simulink model "ASM_Traffic_new"  (R2024a)
settings: Solver=ode1  StartTime=SIM.tstart.v  StopTime=SIM.tend.v  FixedStep=SIM.StepSize.v  RelTol=1e-3
PostLoadFcn:
  | if any(exist('dsrtsu_mdlpostloadfcn', 'file') ~= 0), dsrtsu_mdlpostloadfcn('Execute', bdroot); end
  | try, asm_mdl_postloadfcn(bdroot, 'UpdateModel', 3600); catch, disp(lasterr); end,
InitFcn:
  | , if any(exist('rtifpga_mdlclblib', 'file') ~= 0), rtifpga_mdlclblib('Init', bdroot); end,
  | , if any(exist('dsmpb_private', 'file') ~= 0), dsmpb_private('dsmpb_mdlclblib', 'Init', bdroot); end,
undefined symbols (not defined in the file): _to_, a0b2, ASM_BrakeHydraulics_DemoSystems, ASM_VehicleDynamics_DemoSystems, b98103fe8ad365046cd0, BrakeCircuit, CPT, Crankshaft, DiscIntNeverNeededParam, dsmsi, FinalDriveAssembly, MDL, ModeSignals, Pos_BrakePedal_Maneuver, rad, RefSignals, s_to_rpm, SIM, SoftECU, Suspension, Tire, Transmission
libraries: ASM_Traffic_lib x135, simulink x100, ASM_Utils_lib x77, ASM_VehicleDynamics_lib x70, ASM_Environment_lib x22, dsmpblib x20, dsmsilib x15, MDLD_Utils_lib x10, ASM_BrakeHydraulics_lib x3
(part 57 of 63)

== system ASM_Traffic_new/Environment/Sensors/PlantModel/Object_Sensor_3D/RadarEffects/Sensor2/RadarEffects ==
  Reset[] : Inport
  Sensor_Idx[] : Inport  Port=2
  Sensor_Data[] : Inport  Port=3
  Angle_Vehicle_CoorSys_E[x;y;z][deg] : Inport  Port=4
  Pos_Vehicle_CoorSys_E[x;y;z][m] : Inport  Port=5
  Angle_Sensor_CoorSys_V[x;y;z][deg] : Inport  Port=6
  Pos_Sensor_CoorSys_V[x;y;z][m] : Inport  Port=7
  Enable : EnablePort
  Bus Creator2 : BusCreator  Inputs=10
  Compare To Zero : simulink/Logic and Bit Operations/Compare To Zero  relop=>  OutDataTypeStr=boolean
  MODELDESK_GROUP : ASM_Utils_lib/ModelDeskInterface/MODELDESK_GROUP  MDLDGroup=Object Sensor 3D 2  ASMProperties=struct('Name','MODELDESK_GROUP','Version','1.0','Library','ASM_Utils_lib')
  RADAR_DETECTION_RANGE_2 : ASM_Traffic_lib/Sensors/RadarEffects/RADAR_DETECTION_RANGE  Tag=ASM_SUBCOMPONENT  Sw_Detection_Range_Enable=MDL.Traffic.Sensors.Radar_Detection_Range_2.Sw_Detection_Range_Enable  Const_Signal_Strength_Threshold=MDL.Traffic.Sensors.Radar_Detection_Range_2.Const_Signal_Strength_Threshold  Const_Attenuation=MDL.Traffic.Sensors.Radar_Detection_Range_2.Const_Attenuation  Map_Antenna_Gain=MDL.Traffic.Sensors.Radar_Detection_Range_2.Map_Antenna_Gain  ASMProperties=struct('Name','RADAR_DETECTION_RANGE','Version','1.0','Library','ASM_Traffic_lib')  ASMInstanceName=radar_detection_range  ASMInstanceID=2
      settings: AttributesFormatString=Instance Name: %<ASMInstanceName>\nInstance ID: %<ASMInstanceID>
  RADAR_MEASUREMENT_NOISE_2 : ASM_Traffic_lib/Sensors/RadarEffects/RADAR_MEASUREMENT_NOISE  Tag=ASM_SUBCOMPONENT  Sw_Measurement_Noise_Enable=MDL.Traffic.Sensors.Radar_Measurement_Noise_2.Sw_Measurement_Noise_Enable  Const_StdDev_Distance=MDL.Traffic.Sensors.Radar_Measurement_Noise_2.Const_StdDev_Distance  Const_StdDev_Angle_Hor=MDL.Traffic.Sensors.Radar_Measurement_Noise_2.Const_StdDev_Angle_Hor  Const_StdDev_Angle_Ver=MDL.Traffic.Sensors.Radar_Measurement_Noise_2.Const_StdDev_Angle_Ver  Const_StdDev_Velocity=MDL.Traffic.Sensors.Radar_Measurement_Noise_2.Const_StdDev_Velocity  Const_Seed_Distance=MDL.Traffic.Sensors.Radar_Measurement_Noise_2.Const_Seed_Distance  Const_Seed_Angle_Hor=MDL.Traffic.Sensors.Radar_Measurement_Noise_2.Const_Seed_Angle_Hor  Const_Seed_Angle_Ver=MDL.Traffic.Sensors.Radar_Measurement_Noise_2.Const_Seed_Angle_Ver  Const_Seed_Velocity=MDL.Traffic.Sensors.Radar_Measurement_Noise_2.Const_Seed_Velocity  Const_Output_Dimension_Objects=MDL.Traffic.Sensors.Radar_Measurement_Noise_2.Const_Output_Dimension_Objects  Const_Output_Dimension_Object_Points=MDL.Traffic.Sensors.Radar_Measurement_Noise_2.Const_Output_Dimension_Object_Points  SimStepSize=SIM.StepSize  ASMProperties=struct('Name','RADAR_MEASUREMENT_NOISE','Version','3.0','Library','ASM_Traffic_lib')  ASMInstanceName=radar_measurement_noise  ASMInstanceID=2
      settings: AttributesFormatString=Instance Name: %<ASMInstanceName>\nInstance ID: %<ASMInstanceID>
  RADAR_OUTPUT_SORT_2 : ASM_Traffic_lib/Sensors/RadarEffects/RADAR_OUTPUT_SORT  Tag=ASM_SUBCOMPONENT  Sw_Sort_Enable=MDL.Traffic.Sensors.Radar_Output_Sort_2.Sw_Sort_Enable  Sw_Sort_Attribute=MDL.Traffic.Sensors.Radar_Output_Sort_2.Sw_Sort_Attribute  Sw_Sort_Direction=MDL.Traffic.Sensors.Radar_Output_Sort_2.Sw_Sort_Direction  ASMProperties=struct('Name','RADAR_OUTPUT_SORT','Version','1.0','Library','ASM_Traffic_lib')  ASMInstanceName=radar_output_sort  ASMInstanceID=2
      settings: AttributesFormatString=Instance Name: %<ASMInstanceName>\nInstance ID: %<ASMInstanceID>
  RADAR_RCS_NOISE_2 : ASM_Traffic_lib/Sensors/RadarEffects/RADAR_RCS_NOISE  Tag=ASM_SUBCOMPONENT  Sw_RCS_Noise_Enable=MDL.Traffic.Sensors.Radar_RCS_Noise_2.Sw_RCS_Noise_Enable  Const_StdDev_RCS_Noise=MDL.Traffic.Sensors.Radar_RCS_Noise_2.Const_StdDev_RCS_Noise  Const_Seed_RCS_Noise=MDL.Traffic.Sensors.Radar_RCS_Noise_2.Const_Seed_RCS_Noise  Const_Output_Dimension_Objects=MDL.Traffic.Sensors.Radar_RCS_Noise_2.Const_Output_Dimension_Objects  Const_Output_Dimension_Object_Points=MDL.Traffic.Sensors.Radar_RCS_Noise_2.Const_Output_Dimension_Object_Points  SimStepSize=SIM.StepSize  ASMProperties=struct('Name','RADAR_RCS_NOISE','Version','3.0','Library','ASM_Traffic_lib')  ASMInstanceName=radar_rcs_noise  ASMInstanceID=2
      settings: AttributesFormatString=Instance Name: %<ASMInstanceName>\nInstance ID: %<ASMInstanceID>
  RADAR_REFLECTION_POINTS_2 : ASM_Traffic_lib/Sensors/RadarEffects/RADAR_REFLECTION_POINTS  Const_Output_Dimension_Objects=MDL.Traffic.Sensors.RadarReflectionPoints_2.Const_Output_Dimension_Objects  Const_Output_Dimension_Object_Points=MDL.Traffic.Sensors.RadarReflectionPoints_2.Const_Output_Dimension_Object_Points  ASMProperties=struct('Name','RADAR_REFLECTION_POINTS','Version','1.0','Library','ASM_Traffic_lib')  ASMInstanceName=radar_reflection_points  ASMInstanceID=2
  RADAR_REFLECTION_POINTS_COORDINATES_2 : ASM_Traffic_lib/Sensors/RadarEffects/RADAR_REFLECTION_POINTS_COORDINATES  ASMProperties=struct('Name','RADAR_REFLECTION_POINTS_COORDINATES','Version','1.0','Library','ASM_Traffic_lib')  ASMInstanceName=radar_reflection_points_coordinates  ASMInstanceID=1
  RADAR_RESOLUTION_CELLS_2 : ASM_Traffic_lib/Sensors/RadarEffects/RADAR_RESOLUTION_CELLS  Tag=ASM_SUBCOMPONENT  Sw_Resolution_Cells_Enable=MDL.Traffic.Sensors.Radar_Resolution_Cells_2.Sw_Resolution_Cells_Enable  Sw_Distance_Resolution_Enable=MDL.Traffic.Sensors.Radar_Resolution_Cells_2.Sw_Distance_Resolution_Enable  Sw_Angle_Hor_Resolution_Enable=MDL.Traffic.Sensors.Radar_Resolution_Cells_2.Sw_Angle_Hor_Resolution_Enable  Sw_Angle_Ver_Resolution_Enable=MDL.Traffic.Sensors.Radar_Resolution_Cells_2.Sw_Angle_Ver_Resolution_Enable  Sw_Velocity_Resolution_Enable=MDL.Traffic.Sensors.Radar_Resolution_Cells_2.Sw_Velocity_Resolution_Enable  Const_Distance_Resolution=MDL.Traffic.Sensors.Radar_Resolution_Cells_2.Const_Distance_Resolution  Const_Angle_Hor_Resolution=MDL.Traffic.Sensors.Radar_Resolution_Cells_2.Const_Angle_Hor_Resolution  Const_Angle_Ver_Resolution=MDL.Traffic.Sensors.Radar_Resolution_Cells_2.Const_Angle_Ver_Resolution  Const_Velocity_Resolution=MDL.Traffic.Sensors.Radar_Resolution_Cells_2.Const_Velocity_Resolution  ASMProperties=struct('Name','RADAR_RESOLUTION_CELLS','Version','1.0','Library','ASM_Traffic_lib')  ASMInstanceName=radar_resolution_cells  ASMInstanceID=2
      settings: AttributesFormatString=Instance Name: %<ASMInstanceName>\nInstance ID: %<ASMInstanceID>
  Terminator{1..6,18} (7 alike) : Terminator
  RadarEffect_Signals[] : Outport  OutputWhenDisabled=reset  InitialOutput=[0]  VectorParamsAs1DForOutWhenUnconnected=off
  wires:
  RADAR_DETECTION_RANGE_2/6 -> RADAR_MEASUREMENT_NOISE_2/6
  RADAR_DETECTION_RANGE_2/5 -> RADAR_MEASUREMENT_NOISE_2/5
  RADAR_DETECTION_RANGE_2/4 -> RADAR_MEASUREMENT_NOISE_2/4
  RADAR_DETECTION_RANGE_2/3 -> RADAR_MEASUREMENT_NOISE_2/3
  RADAR_DETECTION_RANGE_2/2 -> RADAR_OUTPUT_SORT_2/1, RADAR_MEASUREMENT_NOISE_2/2
  Reset[]/1 -> RADAR_RCS_NOISE_2/1, RADAR_MEASUREMENT_NOISE_2/1
  RADAR_REFLECTION_POINTS_2/7 -> RADAR_RCS_NOISE_2/3
  RADAR_OUTPUT_SORT_2/6 -> RADAR_REFLECTION_POINTS_COORDINATES_2/8, Bus Creator2/5  "Angle_Ver_CoorSys_S[deg]"
  RADAR_OUTPUT_SORT_2/9 -> Bus Creator2/8  "Object_Type[]"
  RADAR_OUTPUT_SORT_2/5 -> RADAR_REFLECTION_POINTS_COORDINATES_2/7, Bus Creator2/4  "Angle_Hor_CoorSys_S[deg]"
  RADAR_REFLECTION_POINTS_COORDINATES_2/3 -> Bus Creator2/10  "Pos_ObjectPoint_CoorSys_S[x;y;z][m]"
  RADAR_OUTPUT_SORT_2/2 -> Compare To Zero/1, Bus Creator2/1  "ID[]"
  RADAR_OUTPUT_SORT_2/4 -> Bus Creator2/3  "v_CoorSys_S[m|s]"
  RADAR_OUTPUT_SORT_2/7 -> Bus Creator2/6  "RCS[dBm2]"
  RADAR_REFLECTION_POINTS_COORDINATES_2/2 -> Bus Creator2/9  "Pos_ObjectPoint_CoorSys_E[x;y;z][m]"
  RADAR_OUTPUT_SORT_2/8 -> Bus Creator2/7  "Object_ID[]"
  RADAR_OUTPUT_SORT_2/3 -> RADAR_REFLECTION_POINTS_COORDINATES_2/6, Bus Creator2/2  "Dist_CoorSys_S[m]"
  Compare To Zero/1 -> RADAR_REFLECTION_POINTS_COORDINATES_2/5
  RADAR_REFLECTION_POINTS_COORDINATES_2/1 -> Terminator6/1
  Pos_Sensor_CoorSys_V[x;y;z][m]/1 -> RADAR_REFLECTION_POINTS_COORDINATES_2/4
  Angle_Sensor_CoorSys_V[x;y;z][deg]/1 -> RADAR_REFLECTION_POINTS_COORDINATES_2/3
  Pos_Vehicle_CoorSys_E[x;y;z][m]/1 -> RADAR_REFLECTION_POINTS_COORDINATES_2/2
  Angle_Vehicle_CoorSys_E[x;y;z][deg]/1 -> RADAR_REFLECTION_POINTS_COORDINATES_2/1
  Bus Creator2/1 -> RadarEffect_Signals[]/1
  Sensor_Data[]/1 -> RADAR_REFLECTION_POINTS_2/2
  RADAR_RESOLUTION_CELLS_2/5 -> RADAR_DETECTION_RANGE_2/4
  RADAR_RESOLUTION_CELLS_2/8 -> RADAR_DETECTION_RANGE_2/7
  RADAR_MEASUREMENT_NOISE_2/5 -> RADAR_OUTPUT_SORT_2/5
  RADAR_MEASUREMENT_NOISE_2/1 -> Terminator4/1
  RADAR_OUTPUT_SORT_2/1 -> Terminator5/1
  RADAR_REFLECTION_POINTS_2/3 -> RADAR_RESOLUTION_CELLS_2/2
  RADAR_DETECTION_RANGE_2/9 -> RADAR_OUTPUT_SORT_2/8
  RADAR_RESOLUTION_CELLS_2/3 -> RADAR_DETECTION_RANGE_2/2
  RADAR_REFLECTION_POINTS_2/4 -> RADAR_RESOLUTION_CELLS_2/3
  Sensor_Idx[]/1 -> RADAR_REFLECTION_POINTS_2/1
  RADAR_DETECTION_RANGE_2/1 -> Terminator2/1
  RADAR_REFLECTION_POINTS_2/2 -> RADAR_RCS_NOISE_2/2, RADAR_RESOLUTION_CELLS_2/1
  RADAR_DETECTION_RANGE_2/7 -> RADAR_OUTPUT_SORT_2/6
  RADAR_REFLECTION_POINTS_2/9 -> RADAR_RESOLUTION_CELLS_2/8
  RADAR_DETECTION_RANGE_2/8 -> RADAR_OUTPUT_SORT_2/7
  RADAR_RESOLUTION_CELLS_2/1 -> Terminator18/1
  RADAR_REFLECTION_POINTS_2/6 -> RADAR_RESOLUTION_CELLS_2/5
  RADAR_MEASUREMENT_NOISE_2/3 -> RADAR_OUTPUT_SORT_2/3
  RADAR_MEASUREMENT_NOISE_2/4 -> RADAR_OUTPUT_SORT_2/4
  RADAR_RESOLUTION_CELLS_2/9 -> RADAR_DETECTION_RANGE_2/8
  RADAR_REFLECTION_POINTS_2/8 -> RADAR_RESOLUTION_CELLS_2/7
  RADAR_MEASUREMENT_NOISE_2/2 -> RADAR_OUTPUT_SORT_2/2
  RADAR_RESOLUTION_CELLS_2/2 -> RADAR_DETECTION_RANGE_2/1
  RADAR_RESOLUTION_CELLS_2/7 -> RADAR_DETECTION_RANGE_2/6
  RADAR_RESOLUTION_CELLS_2/6 -> RADAR_DETECTION_RANGE_2/5
  RADAR_RCS_NOISE_2/1 -> Terminator1/1
  RADAR_REFLECTION_POINTS_2/5 -> RADAR_RESOLUTION_CELLS_2/4
  RADAR_REFLECTION_POINTS_2/1 -> Terminator3/1
  RADAR_RESOLUTION_CELLS_2/4 -> RADAR_DETECTION_RANGE_2/3
  RADAR_RCS_NOISE_2/2 -> RADAR_RESOLUTION_CELLS_2/6

== system ASM_Traffic_new/Environment/Sensors/PlantModel/Object_Sensor_3D/RadarEffects/Sensor2/RadarEffectsOutput ==
  SensorScheudlingEnable[0|1] : Inport
  SensorActive : Inport  Port=2
  SensorEnable[0|1] : Inport  Port=3
  DelayPulse[0|1] : Inport  Port=4
  RadarEffect_Signals_In[] : Inport  Port=5
  HoldSignals : Subsystem
  Logical Operator2 : Logic  Operator=OR  AllPortsSameDT=off  OutDataTypeStr=boolean
  RADAR_SIGNALS_DELAY_2 : ASM_Traffic_lib/Sensors/RadarEffects/RADAR_SIGNALS_DELAY  ASMProperties=struct('Name','RADAR_SIGNALS_DELAY','Version','1.0','Library','ASM_Traffic_lib')  ASMInstanceName=radar_signals_delay  ASMInstanceID=1
  ResetPulse : Subsystem
  SignalBus : Subsystem
  RadarEffect_Signals_Out[] : Outport  VectorParamsAs1DForOutWhenUnconnected=off
  wires:
  Logical Operator2/1 -> HoldSignals/Enable
  SensorEnable[0|1]/1 -> Logical Operator2/2
  SensorScheudlingEnable[0|1]/1 -> ResetPulse/1(Enable[0|1])
  HoldSignals/1(RadarEffect_Signals_Out[]) -> RADAR_SIGNALS_DELAY_2/3
  RadarEffect_Signals_In[]/1 -> HoldSignals/2(RadarEffect_Signals_In[])
  SensorActive/1 -> ResetPulse/2(SensorActive[0|1])
  DelayPulse[0|1]/1 -> RADAR_SIGNALS_DELAY_2/2
  ResetPulse/1(ResetPulse[0|1]) -> HoldSignals/1(ResetPulse[0|1]), Logical Operator2/1, RADAR_SIGNALS_DELAY_2/1
  SignalBus/1(RadarEffect_Signals_Out[]) -> RadarEffect_Signals_Out[]/1
  RADAR_SIGNALS_DELAY_2/1 -> SignalBus/1(RadarEffect_Signals_In[])

== system ASM_Traffic_new/Environment/Sensors/PlantModel/Object_Sensor_3D/RadarEffects/Sensor3/RadarEffects ==
  Reset[] : Inport
  Sensor_Idx[] : Inport  Port=2
  Sensor_Data[] : Inport  Port=3
  Angle_Vehicle_CoorSys_E[x;y;z][deg] : Inport  Port=4
  Pos_Vehicle_CoorSys_E[x;y;z][m] : Inport  Port=5
  Angle_Sensor_CoorSys_V[x;y;z][deg] : Inport  Port=6
  Pos_Sensor_CoorSys_V[x;y;z][m] : Inport  Port=7
  Enable : EnablePort
  Bus Creator2 : BusCreator  Inputs=10
  Compare To Zero : simulink/Logic and Bit Operations/Compare To Zero  relop=>  OutDataTypeStr=boolean
  MODELDESK_GROUP : ASM_Utils_lib/ModelDeskInterface/MODELDESK_GROUP  MDLDGroup=Object Sensor 3D 3  ASMProperties=struct('Name','MODELDESK_GROUP','Version','1.0','Library','ASM_Utils_lib')
  RADAR_DETECTION_RANGE_3 : ASM_Traffic_lib/Sensors/RadarEffects/RADAR_DETECTION_RANGE  Tag=ASM_SUBCOMPONENT  Sw_Detection_Range_Enable=MDL.Traffic.Sensors.Radar_Detection_Range_3.Sw_Detection_Range_Enable  Const_Signal_Strength_Threshold=MDL.Traffic.Sensors.Radar_Detection_Range_3.Const_Signal_Strength_Threshold  Const_Attenuation=MDL.Traffic.Sensors.Radar_Detection_Range_3.Const_Attenuation  Map_Antenna_Gain=MDL.Traffic.Sensors.Radar_Detection_Range_3.Map_Antenna_Gain  ASMProperties=struct('Name','RADAR_DETECTION_RANGE','Version','1.0','Library','ASM_Traffic_lib')  ASMInstanceName=radar_detection_range  ASMInstanceID=3
      settings: AttributesFormatString=Instance Name: %<ASMInstanceName>\nInstance ID: %<ASMInstanceID>
  RADAR_MEASUREMENT_NOISE_3 : ASM_Traffic_lib/Sensors/RadarEffects/RADAR_MEASUREMENT_NOISE  Tag=ASM_SUBCOMPONENT  Sw_Measurement_Noise_Enable=MDL.Traffic.Sensors.Radar_Measurement_Noise_3.Sw_Measurement_Noise_Enable  Const_StdDev_Distance=MDL.Traffic.Sensors.Radar_Measurement_Noise_3.Const_StdDev_Distance  Const_StdDev_Angle_Hor=MDL.Traffic.Sensors.Radar_Measurement_Noise_3.Const_StdDev_Angle_Hor  Const_StdDev_Angle_Ver=MDL.Traffic.Sensors.Radar_Measurement_Noise_3.Const_StdDev_Angle_Ver  Const_StdDev_Velocity=MDL.Traffic.Sensors.Radar_Measurement_Noise_3.Const_StdDev_Velocity  Const_Seed_Distance=MDL.Traffic.Sensors.Radar_Measurement_Noise_3.Const_Seed_Distance  Const_Seed_Angle_Hor=MDL.Traffic.Sensors.Radar_Measurement_Noise_3.Const_Seed_Angle_Hor  Const_Seed_Angle_Ver=MDL.Traffic.Sensors.Radar_Measurement_Noise_3.Const_Seed_Angle_Ver  Const_Seed_Velocity=MDL.Traffic.Sensors.Radar_Measurement_Noise_3.Const_Seed_Velocity  Const_Output_Dimension_Objects=MDL.Traffic.Sensors.Radar_Measurement_Noise_3.Const_Output_Dimension_Objects  Const_Output_Dimension_Object_Points=MDL.Traffic.Sensors.Radar_Measurement_Noise_3.Const_Output_Dimension_Object_Points  SimStepSize=SIM.StepSize  ASMProperties=struct('Name','RADAR_MEASUREMENT_NOISE','Version','3.0','Library','ASM_Traffic_lib')  ASMInstanceName=radar_measurement_noise  ASMInstanceID=3
      settings: AttributesFormatString=Instance Name: %<ASMInstanceName>\nInstance ID: %<ASMInstanceID>
  RADAR_OUTPUT_SORT_3 : ASM_Traffic_lib/Sensors/RadarEffects/RADAR_OUTPUT_SORT  Tag=ASM_SUBCOMPONENT  Sw_Sort_Enable=MDL.Traffic.Sensors.Radar_Output_Sort_3.Sw_Sort_Enable  Sw_Sort_Attribute=MDL.Traffic.Sensors.Radar_Output_Sort_3.Sw_Sort_Attribute  Sw_Sort_Direction=MDL.Traffic.Sensors.Radar_Output_Sort_3.Sw_Sort_Direction  ASMProperties=struct('Name','RADAR_OUTPUT_SORT','Version','1.0','Library','ASM_Traffic_lib')  ASMInstanceName=radar_output_sort  ASMInstanceID=3
      settings: AttributesFormatString=Instance Name: %<ASMInstanceName>\nInstance ID: %<ASMInstanceID>
  RADAR_RCS_NOISE_3 : ASM_Traffic_lib/Sensors/RadarEffects/RADAR_RCS_NOISE  Tag=ASM_SUBCOMPONENT  Sw_RCS_Noise_Enable=MDL.Traffic.Sensors.Radar_RCS_Noise_3.Sw_RCS_Noise_Enable  Const_StdDev_RCS_Noise=MDL.Traffic.Sensors.Radar_RCS_Noise_3.Const_StdDev_RCS_Noise  Const_Seed_RCS_Noise=MDL.Traffic.Sensors.Radar_RCS_Noise_3.Const_Seed_RCS_Noise  Const_Output_Dimension_Objects=MDL.Traffic.Sensors.Radar_RCS_Noise_3.Const_Output_Dimension_Objects  Const_Output_Dimension_Object_Points=MDL.Traffic.Sensors.Radar_RCS_Noise_3.Const_Output_Dimension_Object_Points  SimStepSize=SIM.StepSize  ASMProperties=struct('Name','RADAR_RCS_NOISE','Version','3.0','Library','ASM_Traffic_lib')  ASMInstanceName=radar_rcs_noise  ASMInstanceID=3
      settings: AttributesFormatString=Instance Name: %<ASMInstanceName>\nInstance ID: %<ASMInstanceID>
  RADAR_REFLECTION_POINTS_3 : ASM_Traffic_lib/Sensors/RadarEffects/RADAR_REFLECTION_POINTS  Const_Output_Dimension_Objects=MDL.Traffic.Sensors.RadarReflectionPoints_3.Const_Output_Dimension_Objects  Const_Output_Dimension_Object_Points=MDL.Traffic.Sensors.RadarReflectionPoints_3.Const_Output_Dimension_Object_Points  ASMProperties=struct('Name','RADAR_REFLECTION_POINTS','Version','1.0','Library','ASM_Traffic_lib')  ASMInstanceName=radar_reflection_points  ASMInstanceID=3
  RADAR_REFLECTION_POINTS_COORDINATES_3 : ASM_Traffic_lib/Sensors/RadarEffects/RADAR_REFLECTION_POINTS_COORDINATES  ASMProperties=struct('Name','RADAR_REFLECTION_POINTS_COORDINATES','Version','1.0','Library','ASM_Traffic_lib')  ASMInstanceName=radar_reflection_points_coordinates  ASMInstanceID=1
  RADAR_RESOLUTION_CELLS_3 : ASM_Traffic_lib/Sensors/RadarEffects/RADAR_RESOLUTION_CELLS  Tag=ASM_SUBCOMPONENT  Sw_Resolution_Cells_Enable=MDL.Traffic.Sensors.Radar_Resolution_Cells_3.Sw_Resolution_Cells_Enable  Sw_Distance_Resolution_Enable=MDL.Traffic.Sensors.Radar_Resolution_Cells_3.Sw_Distance_Resolution_Enable  Sw_Angle_Hor_Resolution_Enable=MDL.Traffic.Sensors.Radar_Resolution_Cells_3.Sw_Angle_Hor_Resolution_Enable  Sw_Angle_Ver_Resolution_Enable=MDL.Traffic.Sensors.Radar_Resolution_Cells_3.Sw_Angle_Ver_Resolution_Enable  Sw_Velocity_Resolution_Enable=MDL.Traffic.Sensors.Radar_Resolution_Cells_3.Sw_Velocity_Resolution_Enable  Const_Distance_Resolution=MDL.Traffic.Sensors.Radar_Resolution_Cells_3.Const_Distance_Resolution  Const_Angle_Hor_Resolution=MDL.Traffic.Sensors.Radar_Resolution_Cells_3.Const_Angle_Hor_Resolution  Const_Angle_Ver_Resolution=MDL.Traffic.Sensors.Radar_Resolution_Cells_3.Const_Angle_Ver_Resolution  Const_Velocity_Resolution=MDL.Traffic.Sensors.Radar_Resolution_Cells_3.Const_Velocity_Resolution  ASMProperties=struct('Name','RADAR_RESOLUTION_CELLS','Version','1.0','Library','ASM_Traffic_lib')  ASMInstanceName=radar_resolution_cells  ASMInstanceID=3
      settings: AttributesFormatString=Instance Name: %<ASMInstanceName>\nInstance ID: %<ASMInstanceID>
  Terminator{1..6,18} (7 alike) : Terminator
  RadarEffect_Signals[] : Outport  OutputWhenDisabled=reset  InitialOutput=[0]  VectorParamsAs1DForOutWhenUnconnected=off
  wires:
  RADAR_DETECTION_RANGE_3/6 -> RADAR_MEASUREMENT_NOISE_3/6
  RADAR_DETECTION_RANGE_3/5 -> RADAR_MEASUREMENT_NOISE_3/5
  RADAR_DETECTION_RANGE_3/4 -> RADAR_MEASUREMENT_NOISE_3/4
  RADAR_DETECTION_RANGE_3/3 -> RADAR_MEASUREMENT_NOISE_3/3
  RADAR_DETECTION_RANGE_3/2 -> RADAR_MEASUREMENT_NOISE_3/2, RADAR_OUTPUT_SORT_3/1
  Reset[]/1 -> RADAR_RCS_NOISE_3/1, RADAR_MEASUREMENT_NOISE_3/1
  RADAR_REFLECTION_POINTS_3/7 -> RADAR_RCS_NOISE_3/3
  RADAR_REFLECTION_POINTS_COORDINATES_3/2 -> Bus Creator2/9  "Pos_ObjectPoint_CoorSys_E[x;y;z][m]"
  RADAR_OUTPUT_SORT_3/7 -> Bus Creator2/6  "RCS[dBm2]"
  RADAR_OUTPUT_SORT_3/9 -> Bus Creator2/8  "Object_Type[]"
  RADAR_OUTPUT_SORT_3/8 -> Bus Creator2/7  "Object_ID[]"
  RADAR_OUTPUT_SORT_3/3 -> RADAR_REFLECTION_POINTS_COORDINATES_3/6, Bus Creator2/2  "Dist_CoorSys_S[m]"
  RADAR_OUTPUT_SORT_3/4 -> Bus Creator2/3  "v_CoorSys_S[m|s]"
  RADAR_OUTPUT_SORT_3/6 -> RADAR_REFLECTION_POINTS_COORDINATES_3/8, Bus Creator2/5  "Angle_Ver_CoorSys_S[deg]"
  RADAR_OUTPUT_SORT_3/5 -> RADAR_REFLECTION_POINTS_COORDINATES_3/7, Bus Creator2/4  "Angle_Hor_CoorSys_S[deg]"
  RADAR_REFLECTION_POINTS_COORDINATES_3/3 -> Bus Creator2/10  "Pos_ObjectPoint_CoorSys_S[x;y;z][m]"
  RADAR_OUTPUT_SORT_3/2 -> Compare To Zero/1, Bus Creator2/1  "ID[]"
  Compare To Zero/1 -> RADAR_REFLECTION_POINTS_COORDINATES_3/5
  Pos_Sensor_CoorSys_V[x;y;z][m]/1 -> RADAR_REFLECTION_POINTS_COORDINATES_3/4
  Angle_Sensor_CoorSys_V[x;y;z][deg]/1 -> RADAR_REFLECTION_POINTS_COORDINATES_3/3
  Pos_Vehicle_CoorSys_E[x;y;z][m]/1 -> RADAR_REFLECTION_POINTS_COORDINATES_3/2
  Angle_Vehicle_CoorSys_E[x;y;z][deg]/1 -> RADAR_REFLECTION_POINTS_COORDINATES_3/1
  RADAR_REFLECTION_POINTS_COORDINATES_3/1 -> Terminator6/1
  Bus Creator2/1 -> RadarEffect_Signals[]/1
  RADAR_MEASUREMENT_NOISE_3/5 -> RADAR_OUTPUT_SORT_3/5
  Sensor_Data[]/1 -> RADAR_REFLECTION_POINTS_3/2
  RADAR_RESOLUTION_CELLS_3/7 -> RADAR_DETECTION_RANGE_3/6
  RADAR_REFLECTION_POINTS_3/9 -> RADAR_RESOLUTION_CELLS_3/8
  RADAR_RESOLUTION_CELLS_3/1 -> Terminator18/1
  RADAR_DETECTION_RANGE_3/8 -> RADAR_OUTPUT_SORT_3/7
  RADAR_RESOLUTION_CELLS_3/6 -> RADAR_DETECTION_RANGE_3/5
  RADAR_OUTPUT_SORT_3/1 -> Terminator5/1
  RADAR_MEASUREMENT_NOISE_3/3 -> RADAR_OUTPUT_SORT_3/3
  RADAR_RCS_NOISE_3/2 -> RADAR_RESOLUTION_CELLS_3/6
  RADAR_MEASUREMENT_NOISE_3/1 -> Terminator4/1
  RADAR_DETECTION_RANGE_3/7 -> RADAR_OUTPUT_SORT_3/6
  RADAR_DETECTION_RANGE_3/9 -> RADAR_OUTPUT_SORT_3/8
  RADAR_REFLECTION_POINTS_3/3 -> RADAR_RESOLUTION_CELLS_3/2
  RADAR_RESOLUTION_CELLS_3/9 -> RADAR_DETECTION_RANGE_3/8
  RADAR_REFLECTION_POINTS_3/5 -> RADAR_RESOLUTION_CELLS_3/4
  RADAR_RESOLUTION_CELLS_3/5 -> RADAR_DETECTION_RANGE_3/4
  RADAR_RESOLUTION_CELLS_3/4 -> RADAR_DETECTION_RANGE_3/3
  RADAR_MEASUREMENT_NOISE_3/2 -> RADAR_OUTPUT_SORT_3/2
  RADAR_REFLECTION_POINTS_3/4 -> RADAR_RESOLUTION_CELLS_3/3
  RADAR_REFLECTION_POINTS_3/8 -> RADAR_RESOLUTION_CELLS_3/7
  RADAR_RESOLUTION_CELLS_3/8 -> RADAR_DETECTION_RANGE_3/7
  RADAR_MEASUREMENT_NOISE_3/4 -> RADAR_OUTPUT_SORT_3/4
  RADAR_DETECTION_RANGE_3/1 -> Terminator2/1
  Sensor_Idx[]/1 -> RADAR_REFLECTION_POINTS_3/1
  RADAR_REFLECTION_POINTS_3/2 -> RADAR_RCS_NOISE_3/2, RADAR_RESOLUTION_CELLS_3/1
  RADAR_RESOLUTION_CELLS_3/2 -> RADAR_DETECTION_RANGE_3/1
  RADAR_REFLECTION_POINTS_3/1 -> Terminator3/1
  RADAR_RCS_NOISE_3/1 -> Terminator1/1
  RADAR_RESOLUTION_CELLS_3/3 -> RADAR_DETECTION_RANGE_3/2
  RADAR_REFLECTION_POINTS_3/6 -> RADAR_RESOLUTION_CELLS_3/5

== system ASM_Traffic_new/Environment/Sensors/PlantModel/Object_Sensor_3D/RadarEffects/Sensor3/RadarEffectsOutput ==
  SensorSchedulingEnable[0|1] : Inport
  SensorActive[0|1] : Inport  Port=2
  SensorEnable[0|1] : Inport  Port=3
  DelayPulse[0|1] : Inport  Port=4
  RadarEffect_Signals_In[] : Inport  Port=5
  HoldSignals : Subsystem
  Logical Operator1 : Logic  Operator=OR  AllPortsSameDT=off  OutDataTypeStr=boolean
  RADAR_SIGNALS_DELAY_3 : ASM_Traffic_lib/Sensors/RadarEffects/RADAR_SIGNALS_DELAY  ASMProperties=struct('Name','RADAR_SIGNALS_DELAY','Version','1.0','Library','ASM_Traffic_lib')  ASMInstanceName=radar_signals_delay  ASMInstanceID=1
  ResetPulse : Subsystem
  SignalBus : Subsystem
  RadarEffect_Signals_Out[] : Outport  VectorParamsAs1DForOutWhenUnconnected=off
  wires:
  SensorEnable[0|1]/1 -> Logical Operator1/2
  SensorActive[0|1]/1 -> ResetPulse/2(SensorActive[0|1])
  HoldSignals/1(RadarEffect_Signals_Out[]) -> RADAR_SIGNALS_DELAY_3/3
  ResetPulse/1(ResetPulse[0|1]) -> HoldSignals/1(ResetPulse[0|1]), Logical Operator1/1, RADAR_SIGNALS_DELAY_3/1
  SensorSchedulingEnable[0|1]/1 -> ResetPulse/1(Enable[0|1])
  Logical Operator1/1 -> HoldSignals/Enable
  SignalBus/1(RadarEffect_Signals_Out[]) -> RadarEffect_Signals_Out[]/1
  RadarEffect_Signals_In[]/1 -> HoldSignals/2(RadarEffect_Signals_In[])
  DelayPulse[0|1]/1 -> RADAR_SIGNALS_DELAY_3/2
  RADAR_SIGNALS_DELAY_3/1 -> SignalBus/1(RadarEffect_Signals_In[])

== system ASM_Traffic_new/Environment/Sensors/UserInterface/DISP_Plant/Object_Sensor_2D/IdxSelect_2DSensor/Scopezone_Element_Data_Selection1 ==
  Scopezone_El_Idx[1_60] : Inport
  Flag_Object_In_Scope[0Out|1In] : Inport  Port=2
  Flag_Sensor_Apex_In_Object[0Out|1In] : Inport  Port=3
  Angle_Hor_Rel[deg] : Inport  Port=4
  Object_ID[] : Inport  Port=5
  Object_Type[] : Inport  Port=6
  Distance[m] : Inport  Port=7
  v_Rel[m|s] : Inport  Port=8
  a_Rel[m|s2] : Inport  Port=9
  Height_Min[m] : Inport  Port=10
  Height_Max[m] : Inport  Port=11
  Angle_Hor_Rel[deg]1 : Subsystem
      mask Display: disp('')
  Distance[m]1 : Subsystem
      mask Display: disp('')
  Flag_Object_In_Scope[0Out|1In]1 : Subsystem
      mask Display: disp('')
  Flag_Sensor_Apex_In_Object[0Out|1In]1 : Subsystem
      mask Display: disp('')
  Height_Max[m]1 : Subsystem
      mask Display: disp('')
  Height_Min[m]1 : Subsystem
      mask Display: disp('')
  Object_ID[]1 : Subsystem
      mask Display: disp('')
  Object_Type[]1 : Subsystem
      mask Display: disp('')
  Selector{3..10} (8 alike) : Selector  InputPortWidth=MDL.Traffic.Sensors.ObjectSensor2D_Calculation.Const_Sensor_Output_Dimension.v  IndexOptions=Index vector (port)  Indices=[1 3]  OutputSizes=1
  Terminator_{1..10} (10 alike) : Terminator
  a_Rel[m|s2]1 : Subsystem
      mask Display: disp('')
  v_Rel[m|s]1 : Subsystem
      mask Display: disp('')
  wires:
  Distance[m]1/1(Out1) -> Terminator_6/1
  v_Rel[m|s]/1 -> Selector7/1
  v_Rel[m|s]1/1(Out1) -> Terminator_7/1
  a_Rel[m|s2]1/1(Out1) -> Terminator_8/1
  Height_Min[m]1/1(Out1) -> Terminator_9/1
  Height_Min[m]/1 -> Selector9/1
  Angle_Hor_Rel[deg]/1 -> Selector3/1
  Distance[m]/1 -> Selector6/1
  Height_Max[m]/1 -> Selector10/1
  Object_Type[]/1 -> Selector5/1
  Object_ID[]1/1(Out1) -> Terminator_3/1
  a_Rel[m|s2]/1 -> Selector8/1
  Angle_Hor_Rel[deg]1/1(Out1) -> Terminator_2/1
  Flag_Sensor_Apex_In_Object[0Out|1In]1/1(Out1) -> Terminator_1/1
  Object_ID[]/1 -> Selector4/1
  Flag_Object_In_Scope[0Out|1In]1/1(Out1) -> Terminator_4/1
  Height_Max[m]1/1(Out1) -> Terminator_10/1
  Flag_Object_In_Scope[0Out|1In]/1 -> Flag_Object_In_Scope[0Out|1In]1/1(In1)
  Scopezone_El_Idx[1_60]/1 -> Selector10/2, Selector9/2, Selector8/2, Selector7/2, Selector6/2, Selector5/2, Selector4/2, Selector3/2
  Selector10/1 -> Height_Max[m]1/1(In1)
  Selector9/1 -> Height_Min[m]1/1(In1)
  Flag_Sensor_Apex_In_Object[0Out|1In]/1 -> Flag_Sensor_Apex_In_Object[0Out|1In]1/1(In1)
  Selector8/1 -> a_Rel[m|s2]1/1(In1)
  Selector7/1 -> v_Rel[m|s]1/1(In1)
  Selector3/1 -> Angle_Hor_Rel[deg]1/1(In1)
  Selector6/1 -> Distance[m]1/1(In1)
  Selector4/1 -> Object_ID[]1/1(In1)
  Object_Type[]1/1(Out1) -> Terminator_5/1
  Selector5/1 -> Object_Type[]1/1(In1)

== system ASM_Traffic_new/Environment/Sensors/UserInterface/DISP_Plant/Object_Sensor_2D/IdxSelect_2DSensor/Scopezone_Element_Data_Selection2 ==
  Scopezone_El_Idx[1_60] : Inport
  Flag_Object_In_Scope[0Out|1In] : Inport  Port=2
  Flag_Sensor_Apex_In_Object[0Out|1In] : Inport  Port=3
  Angle_Hor_Rel[deg] : Inport  Port=4
  Object_ID[] : Inport  Port=5
  Object_Type[] : Inport  Port=6
  Distance[m] : Inport  Port=7
  v_Rel[m|s] : Inport  Port=8
  a_Rel[m|s2] : Inport  Port=9
  Height_Min[m] : Inport  Port=10
  Height_Max[m] : Inport  Port=11
  Angle_Hor_Rel[deg]1 : Subsystem
      mask Display: disp('')
  Distance[m]1 : Subsystem
      mask Display: disp('')
  Flag_Object_In_Scope[0Out|1In]1 : Subsystem
      mask Display: disp('')
  Flag_Sensor_Apex_In_Object[0Out|1In]1 : Subsystem
      mask Display: disp('')
  Height_Max[m]1 : Subsystem
      mask Display: disp('')
  Height_Min[m]1 : Subsystem
      mask Display: disp('')
  Object_ID[]1 : Subsystem
      mask Display: disp('')
  Object_Type[]1 : Subsystem
      mask Display: disp('')
  Selector{3..10} (8 alike) : Selector  InputPortWidth=MDL.Traffic.Sensors.ObjectSensor2D_Calculation.Const_Sensor_Output_Dimension.v  IndexOptions=Index vector (port)  Indices=[1 3]  OutputSizes=1
  Terminator_{1..10} (10 alike) : Terminator
  a_Rel[m|s2]1 : Subsystem
      mask Display: disp('')
  v_Rel[m|s]1 : Subsystem
      mask Display: disp('')
  wires:
  Selector5/1 -> Object_Type[]1/1(In1)
  Object_Type[]1/1(Out1) -> Terminator_5/1
  Selector4/1 -> Object_ID[]1/1(In1)
  Selector6/1 -> Distance[m]1/1(In1)
  Selector3/1 -> Angle_Hor_Rel[deg]1/1(In1)
  Selector7/1 -> v_Rel[m|s]1/1(In1)
  Selector8/1 -> a_Rel[m|s2]1/1(In1)
  Flag_Sensor_Apex_In_Object[0Out|1In]/1 -> Flag_Sensor_Apex_In_Object[0Out|1In]1/1(In1)
  Selector9/1 -> Height_Min[m]1/1(In1)
  Selector10/1 -> Height_Max[m]1/1(In1)
  Scopezone_El_Idx[1_60]/1 -> Selector3/2, Selector4/2, Selector5/2, Selector6/2, Selector7/2, Selector8/2, Selector9/2, Selector10/2
  Flag_Object_In_Scope[0Out|1In]/1 -> Flag_Object_In_Scope[0Out|1In]1/1(In1)
  Height_Max[m]1/1(Out1) -> Terminator_10/1
  Flag_Object_In_Scope[0Out|1In]1/1(Out1) -> Terminator_4/1
  Object_ID[]/1 -> Selector4/1
  Flag_Sensor_Apex_In_Object[0Out|1In]1/1(Out1) -> Terminator_1/1
  Angle_Hor_Rel[deg]1/1(Out1) -> Terminator_2/1
  a_Rel[m|s2]/1 -> Selector8/1
  Object_ID[]1/1(Out1) -> Terminator_3/1
  Object_Type[]/1 -> Selector5/1
  Height_Max[m]/1 -> Selector10/1
  Distance[m]/1 -> Selector6/1
  Angle_Hor_Rel[deg]/1 -> Selector3/1
  Height_Min[m]/1 -> Selector9/1
  Height_Min[m]1/1(Out1) -> Terminator_9/1
  a_Rel[m|s2]1/1(Out1) -> Terminator_8/1
  v_Rel[m|s]1/1(Out1) -> Terminator_7/1
  v_Rel[m|s]/1 -> Selector7/1
  Distance[m]1/1(Out1) -> Terminator_6/1

== system ASM_Traffic_new/Environment/Sensors/UserInterface/DISP_Plant/Object_Sensor_2D/IdxSelect_2DSensor/Scopezone_Element_Data_Selection3 ==
  Scopezone_El_Idx[1_60] : Inport
  Flag_Object_In_Scope[0Out|1In] : Inport  Port=2
  Flag_Sensor_Apex_In_Object[0Out|1In] : Inport  Port=3
  Angle_Hor_Rel[deg] : Inport  Port=4
  Object_ID[] : Inport  Port=5
  Object_Type[] : Inport  Port=6
  Distance[m] : Inport  Port=7
  v_Rel[m|s] : Inport  Port=8
  a_Rel[m|s2] : Inport  Port=9
  Height_Min[m] : Inport  Port=10
  Height_Max[m] : Inport  Port=11
  Angle_Hor_Rel[deg]1 : Subsystem
      mask Display: disp('')
  Distance[m]1 : Subsystem
      mask Display: disp('')
  Flag_Object_In_Scope[0Out|1In]1 : Subsystem
      mask Display: disp('')
  Flag_Sensor_Apex_In_Object[0Out|1In]1 : Subsystem
      mask Display: disp('')
  Height_Max[m]1 : Subsystem
      mask Display: disp('')
  Height_Min[m]1 : Subsystem
      mask Display: disp('')
  Object_ID[]1 : Subsystem
      mask Display: disp('')
  Object_Type[]1 : Subsystem
      mask Display: disp('')
  Selector{3..10} (8 alike) : Selector  InputPortWidth=MDL.Traffic.Sensors.ObjectSensor2D_Calculation.Const_Sensor_Output_Dimension.v  IndexOptions=Index vector (port)  Indices=[1 3]  OutputSizes=1
  Terminator_{1..10} (10 alike) : Terminator
  a_Rel[m|s2]1 : Subsystem
      mask Display: disp('')
  v_Rel[m|s]1 : Subsystem
      mask Display: disp('')
  wires:
  Distance[m]1/1(Out1) -> Terminator_6/1
  v_Rel[m|s]/1 -> Selector7/1
  v_Rel[m|s]1/1(Out1) -> Terminator_7/1
  a_Rel[m|s2]1/1(Out1) -> Terminator_8/1
  Height_Min[m]1/1(Out1) -> Terminator_9/1
  Height_Min[m]/1 -> Selector9/1
  Angle_Hor_Rel[deg]/1 -> Selector3/1
  Distance[m]/1 -> Selector6/1
  Height_Max[m]/1 -> Selector10/1
  Object_Type[]/1 -> Selector5/1
  Object_ID[]1/1(Out1) -> Terminator_3/1
  a_Rel[m|s2]/1 -> Selector8/1
  Angle_Hor_Rel[deg]1/1(Out1) -> Terminator_2/1
  Flag_Sensor_Apex_In_Object[0Out|1In]1/1(Out1) -> Terminator_1/1
  Object_ID[]/1 -> Selector4/1
  Flag_Object_In_Scope[0Out|1In]1/1(Out1) -> Terminator_4/1
  Height_Max[m]1/1(Out1) -> Terminator_10/1
  Flag_Object_In_Scope[0Out|1In]/1 -> Flag_Object_In_Scope[0Out|1In]1/1(In1)
  Scopezone_El_Idx[1_60]/1 -> Selector10/2, Selector9/2, Selector8/2, Selector7/2, Selector6/2, Selector5/2, Selector4/2, Selector3/2
  Selector10/1 -> Height_Max[m]1/1(In1)
  Selector9/1 -> Height_Min[m]1/1(In1)
  Flag_Sensor_Apex_In_Object[0Out|1In]/1 -> Flag_Sensor_Apex_In_Object[0Out|1In]1/1(In1)
  Selector8/1 -> a_Rel[m|s2]1/1(In1)
  Selector7/1 -> v_Rel[m|s]1/1(In1)
  Selector3/1 -> Angle_Hor_Rel[deg]1/1(In1)
  Selector6/1 -> Distance[m]1/1(In1)
  Selector4/1 -> Object_ID[]1/1(In1)
  Object_Type[]1/1(Out1) -> Terminator_5/1
  Selector5/1 -> Object_Type[]1/1(In1)

== system ASM_Traffic_new/Environment/Sensors/UserInterface/DISP_Plant/Object_Sensor_2D/IdxSelect_2DSensor/Scopezone_Element_Data_Selection4 ==
  Scopezone_El_Idx[1_60] : Inport
  Flag_Object_In_Scope[0Out|1In] : Inport  Port=2
  Flag_Sensor_Apex_In_Object[0Out|1In] : Inport  Port=3
  Angle_Hor_Rel[deg] : Inport  Port=4
  Object_ID[] : Inport  Port=5
  Object_Type[] : Inport  Port=6
  Distance[m] : Inport  Port=7
  v_Rel[m|s] : Inport  Port=8
  a_Rel[m|s2] : Inport  Port=9
  Height_Min[m] : Inport  Port=10
  Height_Max[m] : Inport  Port=11
  Angle_Hor_Rel[deg]1 : Subsystem
      mask Display: disp('')
  Distance[m]1 : Subsystem
      mask Display: disp('')
  Flag_Object_In_Scope[0Out|1In]1 : Subsystem
      mask Display: disp('')
  Flag_Sensor_Apex_In_Object[0Out|1In]1 : Subsystem
      mask Display: disp('')
  Height_Max[m]1 : Subsystem
      mask Display: disp('')
  Height_Min[m]1 : Subsystem
      mask Display: disp('')
  Object_ID[]1 : Subsystem
      mask Display: disp('')
  Object_Type[]1 : Subsystem
      mask Display: disp('')
  Selector{3..10} (8 alike) : Selector  InputPortWidth=MDL.Traffic.Sensors.ObjectSensor2D_Calculation.Const_Sensor_Output_Dimension.v  IndexOptions=Index vector (port)  Indices=[1 3]  OutputSizes=1
  Terminator_{1..10} (10 alike) : Terminator
  a_Rel[m|s2]1 : Subsystem
      mask Display: disp('')
  v_Rel[m|s]1 : Subsystem
      mask Display: disp('')
  wires:
  Selector5/1 -> Object_Type[]1/1(In1)
  Object_Type[]1/1(Out1) -> Terminator_5/1
  Selector4/1 -> Object_ID[]1/1(In1)
  Selector6/1 -> Distance[m]1/1(In1)
  Selector3/1 -> Angle_Hor_Rel[deg]1/1(In1)
  Selector7/1 -> v_Rel[m|s]1/1(In1)
  Selector8/1 -> a_Rel[m|s2]1/1(In1)
  Flag_Sensor_Apex_In_Object[0Out|1In]/1 -> Flag_Sensor_Apex_In_Object[0Out|1In]1/1(In1)
  Selector9/1 -> Height_Min[m]1/1(In1)
  Selector10/1 -> Height_Max[m]1/1(In1)
  Scopezone_El_Idx[1_60]/1 -> Selector3/2, Selector4/2, Selector5/2, Selector6/2, Selector7/2, Selector8/2, Selector9/2, Selector10/2
  Flag_Object_In_Scope[0Out|1In]/1 -> Flag_Object_In_Scope[0Out|1In]1/1(In1)
  Height_Max[m]1/1(Out1) -> Terminator_10/1
  Flag_Object_In_Scope[0Out|1In]1/1(Out1) -> Terminator_4/1
  Object_ID[]/1 -> Selector4/1
  Flag_Sensor_Apex_In_Object[0Out|1In]1/1(Out1) -> Terminator_1/1
  Angle_Hor_Rel[deg]1/1(Out1) -> Terminator_2/1
  a_Rel[m|s2]/1 -> Selector8/1
  Object_ID[]1/1(Out1) -> Terminator_3/1
  Object_Type[]/1 -> Selector5/1
  Height_Max[m]/1 -> Selector10/1
  Distance[m]/1 -> Selector6/1
  Angle_Hor_Rel[deg]/1 -> Selector3/1
  Height_Min[m]/1 -> Selector9/1
  Height_Min[m]1/1(Out1) -> Terminator_9/1
  a_Rel[m|s2]1/1(Out1) -> Terminator_8/1
  v_Rel[m|s]1/1(Out1) -> Terminator_7/1
  v_Rel[m|s]/1 -> Selector7/1
  Distance[m]1/1(Out1) -> Terminator_6/1

== system ASM_Traffic_new/Environment/Sensors/UserInterface/DISP_Plant/Object_Sensor_2D/IdxSelect_2DSensor/Scopezone_Element_Data_Selection5 ==
  Scopezone_El_Idx[1_60] : Inport
  Flag_Object_In_Scope[0Out|1In] : Inport  Port=2
  Flag_Sensor_Apex_In_Object[0Out|1In] : Inport  Port=3
  Angle_Hor_Rel[deg] : Inport  Port=4
  Object_ID[] : Inport  Port=5
  Object_Type[] : Inport  Port=6
  Distance[m] : Inport  Port=7
  v_Rel[m|s] : Inport  Port=8
  a_Rel[m|s2] : Inport  Port=9
  Height_Min[m] : Inport  Port=10
  Height_Max[m] : Inport  Port=11
  Angle_Hor_Rel[deg]1 : Subsystem
      mask Display: disp('')
  Distance[m]1 : Subsystem
      mask Display: disp('')
  Flag_Object_In_Scope[0Out|1In]1 : Subsystem
      mask Display: disp('')
  Flag_Sensor_Apex_In_Object[0Out|1In]1 : Subsystem
      mask Display: disp('')
  Height_Max[m]1 : Subsystem
      mask Display: disp('')
  Height_Min[m]1 : Subsystem
      mask Display: disp('')
  Object_ID[]1 : Subsystem
      mask Display: disp('')
  Object_Type[]1 : Subsystem
      mask Display: disp('')
  Selector{3..10} (8 alike) : Selector  InputPortWidth=MDL.Traffic.Sensors.ObjectSensor2D_Calculation.Const_Sensor_Output_Dimension.v  IndexOptions=Index vector (port)  Indices=[1 3]  OutputSizes=1
  Terminator_{1..10} (10 alike) : Terminator
  a_Rel[m|s2]1 : Subsystem
      mask Display: disp('')
  v_Rel[m|s]1 : Subsystem
      mask Display: disp('')
  wires:
  Distance[m]1/1(Out1) -> Terminator_6/1
  v_Rel[m|s]/1 -> Selector7/1
  v_Rel[m|s]1/1(Out1) -> Terminator_7/1
  a_Rel[m|s2]1/1(Out1) -> Terminator_8/1
  Height_Min[m]1/1(Out1) -> Terminator_9/1
  Height_Min[m]/1 -> Selector9/1
  Angle_Hor_Rel[deg]/1 -> Selector3/1
  Distance[m]/1 -> Selector6/1
  Height_Max[m]/1 -> Selector10/1
  Object_Type[]/1 -> Selector5/1
  Object_ID[]1/1(Out1) -> Terminator_3/1
  a_Rel[m|s2]/1 -> Selector8/1
  Angle_Hor_Rel[deg]1/1(Out1) -> Terminator_2/1
  Flag_Sensor_Apex_In_Object[0Out|1In]1/1(Out1) -> Terminator_1/1
  Object_ID[]/1 -> Selector4/1
  Flag_Object_In_Scope[0Out|1In]1/1(Out1) -> Terminator_4/1
  Height_Max[m]1/1(Out1) -> Terminator_10/1
  Flag_Object_In_Scope[0Out|1In]/1 -> Flag_Object_In_Scope[0Out|1In]1/1(In1)
  Scopezone_El_Idx[1_60]/1 -> Selector10/2, Selector9/2, Selector8/2, Selector7/2, Selector6/2, Selector5/2, Selector4/2, Selector3/2
  Selector10/1 -> Height_Max[m]1/1(In1)
  Selector9/1 -> Height_Min[m]1/1(In1)
  Flag_Sensor_Apex_In_Object[0Out|1In]/1 -> Flag_Sensor_Apex_In_Object[0Out|1In]1/1(In1)
  Selector8/1 -> a_Rel[m|s2]1/1(In1)
  Selector7/1 -> v_Rel[m|s]1/1(In1)
  Selector3/1 -> Angle_Hor_Rel[deg]1/1(In1)
  Selector6/1 -> Distance[m]1/1(In1)
  Selector4/1 -> Object_ID[]1/1(In1)
  Object_Type[]1/1(Out1) -> Terminator_5/1
  Selector5/1 -> Object_Type[]1/1(In1)

== system ASM_Traffic_new/Environment/Sensors/UserInterface/DISP_Plant/Object_Sensor_2D/Object_Sensor_2D_VisualizationData/Sensor_1_Front_Long ==
  Sensor : Inport
  Angle_Hor_Rel[deg] : Gain
  Angle_ScopeZone_Horizontal[deg] : Gain
  Angle_z_Orientation_Sensor_CoorSys_V[deg] : Gain
  Bus Selector : BusSelector  OutputSignals=Parameters.Sensor_Enable[0Off|1On],Parameters.Sensor_Detection_Mode[1Ray|2Sector],Parameters.Length_ScopeZone[m],Parameters.Pos_Sensor_Apex_CoorSys_V[x;y;z][m],Parameters.Angle_z_Orientation_Sensor_CoorSys_V[deg],Parameters.Angle_ScopeZone_Horizontal[deg],Parameters.SensorIdx[],SensorOutput.Object_ID[],SensorOutput.Distance[m],SensorOutput.Angle_Hor_Rel[deg]
  Distance[m] : Gain
  Length_ScopeZone[m] : Gain
  Object_ID[] : Gain
  Pos_Sensor_Apex_CoorSys_V[x;y;z][m] : Gain
  SensorIdx[] : Gain
  Sensor_Detection_Mode[1Ray|2Sector] : Gain
  Sensor_Enable[0Off|1On] : Gain
  Terminator{,1..9} (10 alike) : Terminator
  wires:
  Sensor/1 -> Bus Selector/1
  Bus Selector/1 -> Sensor_Enable[0Off|1On]/1  "<Sensor_Enable[0Off|1On]>"
  Sensor_Enable[0Off|1On]/1 -> Terminator/1
  Sensor_Detection_Mode[1Ray|2Sector]/1 -> Terminator1/1
  Bus Selector/2 -> Sensor_Detection_Mode[1Ray|2Sector]/1  "<Sensor_Detection_Mode[1Ray|2Sector]>"
  Pos_Sensor_Apex_CoorSys_V[x;y;z][m]/1 -> Terminator2/1
  Angle_z_Orientation_Sensor_CoorSys_V[deg]/1 -> Terminator3/1
  Angle_ScopeZone_Horizontal[deg]/1 -> Terminator4/1
  SensorIdx[]/1 -> Terminator5/1
  Object_ID[]/1 -> Terminator6/1
  Distance[m]/1 -> Terminator7/1
  Angle_Hor_Rel[deg]/1 -> Terminator8/1
  Bus Selector/4 -> Pos_Sensor_Apex_CoorSys_V[x;y;z][m]/1  "<Pos_Sensor_Apex_CoorSys_V[x;y;z][m]>"
  Bus Selector/5 -> Angle_z_Orientation_Sensor_CoorSys_V[deg]/1  "<Angle_z_Orientation_Sensor_CoorSys_V[deg]>"
  Bus Selector/6 -> Angle_ScopeZone_Horizontal[deg]/1  "<Angle_ScopeZone_Horizontal[deg]>"
  Bus Selector/7 -> SensorIdx[]/1  "<SensorIdx[]>"
  Bus Selector/8 -> Object_ID[]/1  "<Object_ID[]>"
  Bus Selector/9 -> Distance[m]/1  "<Distance[m]>"
  Bus Selector/10 -> Angle_Hor_Rel[deg]/1  "<Angle_Hor_Rel[deg]>"
  Length_ScopeZone[m]/1 -> Terminator9/1
  Bus Selector/3 -> Length_ScopeZone[m]/1  "<Length_ScopeZone[m]>"

== system ASM_Traffic_new/Environment/Sensors/UserInterface/DISP_Plant/Object_Sensor_2D/Object_Sensor_2D_VisualizationData/Sensor_2_Front_Left ==
  Sensor : Inport
  Angle_Hor_Rel[deg] : Gain
  Angle_ScopeZone_Horizontal[deg] : Gain
  Angle_z_Orientation_Sensor_CoorSys_V[deg] : Gain
  Bus Selector : BusSelector  OutputSignals=Parameters.Sensor_Enable[0Off|1On],Parameters.Sensor_Detection_Mode[1Ray|2Sector],Parameters.Length_ScopeZone[m],Parameters.Pos_Sensor_Apex_CoorSys_V[x;y;z][m],Parameters.Angle_z_Orientation_Sensor_CoorSys_V[deg],Parameters.Angle_ScopeZone_Horizontal[deg],Parameters.SensorIdx[],SensorOutput.Object_ID[],SensorOutput.Distance[m],SensorOutput.Angle_Hor_Rel[deg]
  Distance[m] : Gain
  Length_ScopeZone[m] : Gain
  Object_ID[] : Gain
  Pos_Sensor_Apex_CoorSys_V[x;y;z][m] : Gain
  SensorIdx[] : Gain
  Sensor_Detection_Mode[1Ray|2Sector] : Gain
  Sensor_Enable[0Off|1On] : Gain
  Terminator{,1..9} (10 alike) : Terminator
  wires:
  Bus Selector/3 -> Length_ScopeZone[m]/1  "<Length_ScopeZone[m]>"
  Length_ScopeZone[m]/1 -> Terminator9/1
  Bus Selector/10 -> Angle_Hor_Rel[deg]/1  "<Angle_Hor_Rel[deg]>"
  Bus Selector/9 -> Distance[m]/1  "<Distance[m]>"
  Bus Selector/8 -> Object_ID[]/1  "<Object_ID[]>"
  Bus Selector/7 -> SensorIdx[]/1  "<SensorIdx[]>"
  Bus Selector/6 -> Angle_ScopeZone_Horizontal[deg]/1  "<Angle_ScopeZone_Horizontal[deg]>"
  Bus Selector/5 -> Angle_z_Orientation_Sensor_CoorSys_V[deg]/1  "<Angle_z_Orientation_Sensor_CoorSys_V[deg]>"
  Bus Selector/4 -> Pos_Sensor_Apex_CoorSys_V[x;y;z][m]/1  "<Pos_Sensor_Apex_CoorSys_V[x;y;z][m]>"
  Angle_Hor_Rel[deg]/1 -> Terminator8/1
  Distance[m]/1 -> Terminator7/1
  Object_ID[]/1 -> Terminator6/1
  SensorIdx[]/1 -> Terminator5/1
  Angle_ScopeZone_Horizontal[deg]/1 -> Terminator4/1
  Angle_z_Orientation_Sensor_CoorSys_V[deg]/1 -> Terminator3/1
  Pos_Sensor_Apex_CoorSys_V[x;y;z][m]/1 -> Terminator2/1
  Bus Selector/2 -> Sensor_Detection_Mode[1Ray|2Sector]/1  "<Sensor_Detection_Mode[1Ray|2Sector]>"
  Sensor_Detection_Mode[1Ray|2Sector]/1 -> Terminator1/1
  Sensor_Enable[0Off|1On]/1 -> Terminator/1
  Bus Selector/1 -> Sensor_Enable[0Off|1On]/1  "<Sensor_Enable[0Off|1On]>"
  Sensor/1 -> Bus Selector/1

== system ASM_Traffic_new/Environment/Sensors/UserInterface/DISP_Plant/Object_Sensor_2D/Object_Sensor_2D_VisualizationData/Sensor_3_Left ==
  Sensor : Inport
  Angle_Hor_Rel[deg] : Gain
  Angle_ScopeZone_Horizontal[deg] : Gain
  Angle_z_Orientation_Sensor_CoorSys_V[deg] : Gain
  Bus Selector : BusSelector  OutputSignals=Parameters.Sensor_Enable[0Off|1On],Parameters.Sensor_Detection_Mode[1Ray|2Sector],Parameters.Length_ScopeZone[m],Parameters.Pos_Sensor_Apex_CoorSys_V[x;y;z][m],Parameters.Angle_z_Orientation_Sensor_CoorSys_V[deg],Parameters.Angle_ScopeZone_Horizontal[deg],Parameters.SensorIdx[],SensorOutput.Object_ID[],SensorOutput.Distance[m],SensorOutput.Angle_Hor_Rel[deg]
  Distance[m] : Gain
  Length_ScopeZone[m] : Gain
  Object_ID[] : Gain
  Pos_Sensor_Apex_CoorSys_V[x;y;z][m] : Gain
  SensorIdx[] : Gain
  Sensor_Detection_Mode[1Ray|2Sector] : Gain
  Sensor_Enable[0Off|1On] : Gain
  Terminator{,1..9} (10 alike) : Terminator
  wires:
  Sensor/1 -> Bus Selector/1
  Bus Selector/1 -> Sensor_Enable[0Off|1On]/1  "<Sensor_Enable[0Off|1On]>"
  Sensor_Enable[0Off|1On]/1 -> Terminator/1
  Sensor_Detection_Mode[1Ray|2Sector]/1 -> Terminator1/1
  Bus Selector/2 -> Sensor_Detection_Mode[1Ray|2Sector]/1  "<Sensor_Detection_Mode[1Ray|2Sector]>"
  Pos_Sensor_Apex_CoorSys_V[x;y;z][m]/1 -> Terminator2/1
  Angle_z_Orientation_Sensor_CoorSys_V[deg]/1 -> Terminator3/1
  Angle_ScopeZone_Horizontal[deg]/1 -> Terminator4/1
  SensorIdx[]/1 -> Terminator5/1
  Object_ID[]/1 -> Terminator6/1
  Distance[m]/1 -> Terminator7/1
  Angle_Hor_Rel[deg]/1 -> Terminator8/1
  Bus Selector/4 -> Pos_Sensor_Apex_CoorSys_V[x;y;z][m]/1  "<Pos_Sensor_Apex_CoorSys_V[x;y;z][m]>"
  Bus Selector/5 -> Angle_z_Orientation_Sensor_CoorSys_V[deg]/1  "<Angle_z_Orientation_Sensor_CoorSys_V[deg]>"
  Bus Selector/6 -> Angle_ScopeZone_Horizontal[deg]/1  "<Angle_ScopeZone_Horizontal[deg]>"
  Bus Selector/7 -> SensorIdx[]/1  "<SensorIdx[]>"
  Bus Selector/8 -> Object_ID[]/1  "<Object_ID[]>"
  Bus Selector/9 -> Distance[m]/1  "<Distance[m]>"
  Bus Selector/10 -> Angle_Hor_Rel[deg]/1  "<Angle_Hor_Rel[deg]>"
  Length_ScopeZone[m]/1 -> Terminator9/1
  Bus Selector/3 -> Length_ScopeZone[m]/1  "<Length_ScopeZone[m]>"

== system ASM_Traffic_new/Environment/Sensors/UserInterface/DISP_Plant/Object_Sensor_2D/Object_Sensor_2D_VisualizationData/Sensor_4_Rear_Left ==
  Sensor : Inport
  Angle_Hor_Rel[deg] : Gain
  Angle_ScopeZone_Horizontal[deg] : Gain
  Angle_z_Orientation_Sensor_CoorSys_V[deg] : Gain
  Bus Selector : BusSelector  OutputSignals=Parameters.Sensor_Enable[0Off|1On],Parameters.Sensor_Detection_Mode[1Ray|2Sector],Parameters.Length_ScopeZone[m],Parameters.Pos_Sensor_Apex_CoorSys_V[x;y;z][m],Parameters.Angle_z_Orientation_Sensor_CoorSys_V[deg],Parameters.Angle_ScopeZone_Horizontal[deg],Parameters.SensorIdx[],SensorOutput.Object_ID[],SensorOutput.Distance[m],SensorOutput.Angle_Hor_Rel[deg]
  Distance[m] : Gain
  Length_ScopeZone[m] : Gain
  Object_ID[] : Gain
  Pos_Sensor_Apex_CoorSys_V[x;y;z][m] : Gain
  SensorIdx[] : Gain
  Sensor_Detection_Mode[1Ray|2Sector] : Gain
  Sensor_Enable[0Off|1On] : Gain
  Terminator{,1..9} (10 alike) : Terminator
  wires:
  Bus Selector/3 -> Length_ScopeZone[m]/1  "<Length_ScopeZone[m]>"
  Length_ScopeZone[m]/1 -> Terminator9/1
  Bus Selector/10 -> Angle_Hor_Rel[deg]/1  "<Angle_Hor_Rel[deg]>"
  Bus Selector/9 -> Distance[m]/1  "<Distance[m]>"
  Bus Selector/8 -> Object_ID[]/1  "<Object_ID[]>"
  Bus Selector/7 -> SensorIdx[]/1  "<SensorIdx[]>"
  Bus Selector/6 -> Angle_ScopeZone_Horizontal[deg]/1  "<Angle_ScopeZone_Horizontal[deg]>"
  Bus Selector/5 -> Angle_z_Orientation_Sensor_CoorSys_V[deg]/1  "<Angle_z_Orientation_Sensor_CoorSys_V[deg]>"
  Bus Selector/4 -> Pos_Sensor_Apex_CoorSys_V[x;y;z][m]/1  "<Pos_Sensor_Apex_CoorSys_V[x;y;z][m]>"
  Angle_Hor_Rel[deg]/1 -> Terminator8/1
  Distance[m]/1 -> Terminator7/1
  Object_ID[]/1 -> Terminator6/1
  SensorIdx[]/1 -> Terminator5/1
  Angle_ScopeZone_Horizontal[deg]/1 -> Terminator4/1
  Angle_z_Orientation_Sensor_CoorSys_V[deg]/1 -> Terminator3/1
  Pos_Sensor_Apex_CoorSys_V[x;y;z][m]/1 -> Terminator2/1
  Bus Selector/2 -> Sensor_Detection_Mode[1Ray|2Sector]/1  "<Sensor_Detection_Mode[1Ray|2Sector]>"
  Sensor_Detection_Mode[1Ray|2Sector]/1 -> Terminator1/1
  Sensor_Enable[0Off|1On]/1 -> Terminator/1
  Bus Selector/1 -> Sensor_Enable[0Off|1On]/1  "<Sensor_Enable[0Off|1On]>"
  Sensor/1 -> Bus Selector/1

== system ASM_Traffic_new/Environment/Sensors/UserInterface/DISP_Plant/Object_Sensor_2D/Object_Sensor_2D_VisualizationData/Sensor_5_Front_Right ==
  Sensor : Inport
  Angle_Hor_Rel[deg] : Gain
  Angle_ScopeZone_Horizontal[deg] : Gain
  Angle_z_Orientation_Sensor_CoorSys_V[deg] : Gain
  Bus Selector : BusSelector  OutputSignals=Parameters.Sensor_Enable[0Off|1On],Parameters.Sensor_Detection_Mode[1Ray|2Sector],Parameters.Length_ScopeZone[m],Parameters.Pos_Sensor_Apex_CoorSys_V[x;y;z][m],Parameters.Angle_z_Orientation_Sensor_CoorSys_V[deg],Parameters.Angle_ScopeZone_Horizontal[deg],Parameters.SensorIdx[],SensorOutput.Object_ID[],SensorOutput.Distance[m],SensorOutput.Angle_Hor_Rel[deg]
  Distance[m] : Gain
  Length_ScopeZone[m] : Gain
  Object_ID[] : Gain
  Pos_Sensor_Apex_CoorSys_V[x;y;z][m] : Gain
  SensorIdx[] : Gain
  Sensor_Detection_Mode[1Ray|2Sector] : Gain
  Sensor_Enable[0Off|1On] : Gain
  Terminator{,1..9} (10 alike) : Terminator
  wires:
  Sensor/1 -> Bus Selector/1
  Bus Selector/1 -> Sensor_Enable[0Off|1On]/1  "<Sensor_Enable[0Off|1On]>"
  Sensor_Enable[0Off|1On]/1 -> Terminator/1
  Sensor_Detection_Mode[1Ray|2Sector]/1 -> Terminator1/1
  Bus Selector/2 -> Sensor_Detection_Mode[1Ray|2Sector]/1  "<Sensor_Detection_Mode[1Ray|2Sector]>"
  Pos_Sensor_Apex_CoorSys_V[x;y;z][m]/1 -> Terminator2/1
  Angle_z_Orientation_Sensor_CoorSys_V[deg]/1 -> Terminator3/1
  Angle_ScopeZone_Horizontal[deg]/1 -> Terminator4/1
  SensorIdx[]/1 -> Terminator5/1
  Object_ID[]/1 -> Terminator6/1
  Distance[m]/1 -> Terminator7/1
  Angle_Hor_Rel[deg]/1 -> Terminator8/1
  Bus Selector/4 -> Pos_Sensor_Apex_CoorSys_V[x;y;z][m]/1  "<Pos_Sensor_Apex_CoorSys_V[x;y;z][m]>"
  Bus Selector/5 -> Angle_z_Orientation_Sensor_CoorSys_V[deg]/1  "<Angle_z_Orientation_Sensor_CoorSys_V[deg]>"
  Bus Selector/6 -> Angle_ScopeZone_Horizontal[deg]/1  "<Angle_ScopeZone_Horizontal[deg]>"
  Bus Selector/7 -> SensorIdx[]/1  "<SensorIdx[]>"
  Bus Selector/8 -> Object_ID[]/1  "<Object_ID[]>"
  Bus Selector/9 -> Distance[m]/1  "<Distance[m]>"
  Bus Selector/10 -> Angle_Hor_Rel[deg]/1  "<Angle_Hor_Rel[deg]>"
  Length_ScopeZone[m]/1 -> Terminator9/1
  Bus Selector/3 -> Length_ScopeZone[m]/1  "<Length_ScopeZone[m]>"
